simulink model "scheme_L2"  (R2025b)
settings: Solver=ode45  StartTime=0.0  StopTime=12  MaxStep=.001  RelTol=1e-8  AbsTol=1e-10

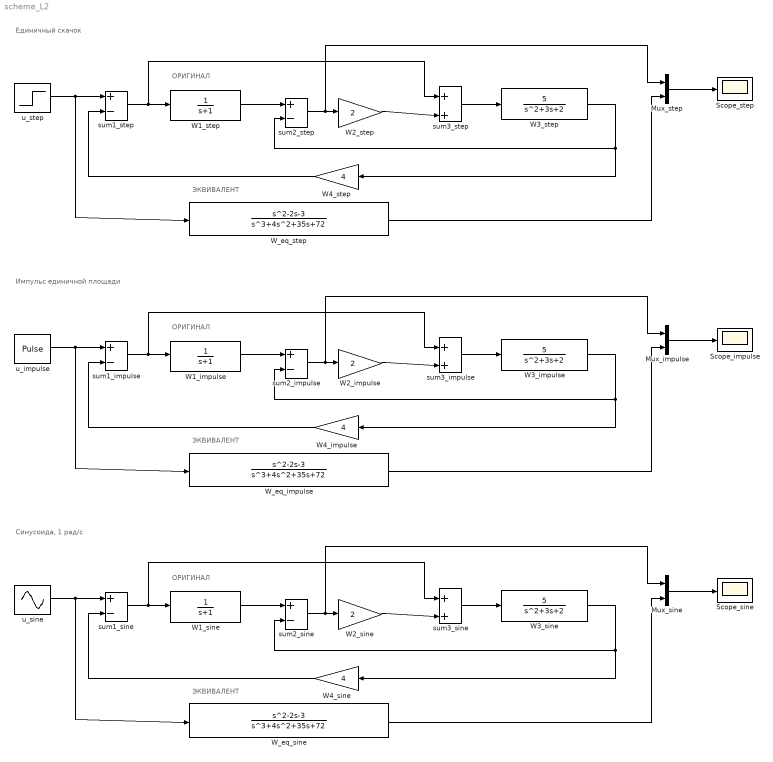
== system scheme_L2 ==
  note: Единичный скачок
  note: ОРИГИНАЛ
  note: ЭКВИВАЛЕНТ
  note: Импульс единичной площади
  note: ОРИГИНАЛ
  note: ЭКВИВАЛЕНТ
  note: Синусоида, 1 рад/с
  note: ОРИГИНАЛ
  note: ЭКВИВАЛЕНТ
  Mux_impulse : Mux  Inputs=2
  Mux_sine : Mux  Inputs=2
  Mux_step : Mux  Inputs=2
  Scope_impulse : Scope
  Scope_sine : Scope
  Scope_step : Scope
  W1_impulse : TransferFcn  Denominator=[1 1]
  W1_sine : TransferFcn  Denominator=[1 1]
  W1_step : TransferFcn  Denominator=[1 1]
  W4_impulse : Gain  Gain=4
  W2_impulse : Gain  Gain=2
  W4_sine : Gain  Gain=4
  W2_sine : Gain  Gain=2
  W4_step : Gain  Gain=4
  W2_step : Gain  Gain=2
  W3_impulse : TransferFcn  Numerator=[5]  Denominator=[1 3 2]
  W3_sine : TransferFcn  Numerator=[5]  Denominator=[1 3 2]
  W3_step : TransferFcn  Numerator=[5]  Denominator=[1 3 2]
  W_eq_impulse : TransferFcn  Numerator=[1 -2 -3]  Denominator=[1 4 35 72]
  W_eq_sine : TransferFcn  Numerator=[1 -2 -3]  Denominator=[1 4 35 72]
  W_eq_step : TransferFcn  Numerator=[1 -2 -3]  Denominator=[1 4 35 72]
  sum1_impulse : Sum  Inputs=+-
  sum1_sine : Sum  Inputs=+-
  sum1_step : Sum  Inputs=+-
  sum2_impulse : Sum  Inputs=+-
  sum2_sine : Sum  Inputs=+-
  sum2_step : Sum  Inputs=+-
  sum3_impulse : Sum  Inputs=++
  sum3_sine : Sum  Inputs=++
  sum3_step : Sum  Inputs=++
  u_impulse : DiscretePulseGenerator  PulseType=Time based  Amplitude=50  Period=20  PulseWidth=0.1  PhaseDelay=0
  u_sine : Sin  Frequency=1  SampleTime=0  Amplitude=1  Phase=0
  u_step : Step  SampleTime=0  Time=0  Before=0  After=1
  wires:
  u_step/1 -> sum1_step/1, W_eq_step/1
  sum1_step/1 -> W1_step/1, sum3_step/1
  W1_step/1 -> sum2_step/1
  sum2_step/1 -> W2_step/1, Mux_step/1
  W2_step/1 -> sum3_step/2
  sum3_step/1 -> W3_step/1
  W3_step/1 -> sum2_step/2, W4_step/1
  W4_step/1 -> sum1_step/2
  W_eq_step/1 -> Mux_step/2
  Mux_step/1 -> Scope_step/1
  u_impulse/1 -> sum1_impulse/1, W_eq_impulse/1
  sum1_impulse/1 -> W1_impulse/1, sum3_impulse/1
  W1_impulse/1 -> sum2_impulse/1
  sum2_impulse/1 -> W2_impulse/1, Mux_impulse/1
  W2_impulse/1 -> sum3_impulse/2
  sum3_impulse/1 -> W3_impulse/1
  W3_impulse/1 -> sum2_impulse/2, W4_impulse/1
  W4_impulse/1 -> sum1_impulse/2
  W_eq_impulse/1 -> Mux_impulse/2
  Mux_impulse/1 -> Scope_impulse/1
  u_sine/1 -> sum1_sine/1, W_eq_sine/1
  sum1_sine/1 -> W1_sine/1, sum3_sine/1
  W1_sine/1 -> sum2_sine/1
  sum2_sine/1 -> W2_sine/1, Mux_sine/1
  W2_sine/1 -> sum3_sine/2
  sum3_sine/1 -> W3_sine/1
  W3_sine/1 -> sum2_sine/2, W4_sine/1
  W4_sine/1 -> sum1_sine/2
  W_eq_sine/1 -> Mux_sine/2
  Mux_sine/1 -> Scope_sine/1
